simulink model "sf_traffic_light"  (R2025b)
settings: Solver=FixedStepDiscrete  StartTime=0.0  StopTime=1000  FixedStep=0.1  RelTol=1e-3  EnableMultiTasking=on
undefined symbols (not defined in the file or in its folder): greenLightLocked, greenLightRequested
libraries: sf_traffic_light_lib x7
settings Model: Creator=The MathWorks, Inc.  LastModifiedBy=The MathWorks, Inc.
settings SolverCC: AlgebraicLoopSolver=TrustRegion
settings DataIOCC: LimitDataPoints=on  SaveFormat=Array  ReturnWorkspaceOutputs=off
settings OptimizationCC: ReuseModelBlockBuffer=off  ExpressionDepthLimit=2147483647.0  InitFltsAndDblsToZero=on  EfficientMapNaN2IntZero=off  LifeSpan=inf
settings DebuggingCC: SaveWithParameterizedLinksMsg=none  UnderspecifiedInitializationDetection=Classic  MergeDetectMultiDrivingBlocksExec=none  SignalResolutionControl=TryResolveAllWithWarning  SolverPrmCheckMsg=warning  MultiTaskDSMMsg=warning  MultiTaskCondExecSysMsg=none  FcnCallInpInsideContextMsg=warning  UnconnectedInputMsg=warning  UnconnectedOutputMsg=warning  UnconnectedLineMsg=warning  StateNameClashWarn=warning  SFUnexpectedBacktrackingDiag=warning  SFNoUnconditionalDefaultTransitionDiag=warning  SFExecutionAtInitializationDiag=none  ArithmeticOperatorsInVariantConditions=warning
settings HardwareCC: ProdBitPerPointer=32.0  ProdBitPerSizeT=32.0  ProdBitPerPtrDiffT=32.0  ProdLargestAtomicFloat=None  ProdIntDivRoundTo=Undefined  ProdEndianess=Unspecified  ProdWordSize=32.0  ProdHWDeviceType=32-bit Generic
settings ModelReferenceCC: EnableRefExpFcnMdlSchedulingChecks=on  PropagateSignalLabelsOutOfModel=off
settings SFSimCC: SimUseLocalCustomCode=off  SimParseCustomCode=off  CustomCodeUndefinedFunction=UseInterfaceOnly
settings RTWCC: RTWUseLocalCustomCode=off  GPUComputeCapability=3.5
settings CodeAppCC: StateflowObjectComments=on
settings GRTTargetCC: TargetFcnLib=ansi_tfl_tmw.mat  TargetLangStandard=C89/C90 (ANSI)  CombineOutputUpdateFcns=off  GRTInterface=on
settings ConfigComp: CovMetricSettings=dw  CovSaveCumulativeToWorkspaceVar=on  CovSaveSingleToWorkspaceVar=on  CovExternalEMLEnable=off  CovSFcnEnable=off

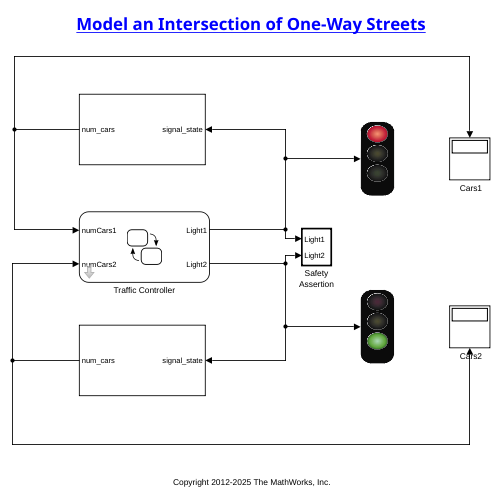
[thumbnail: Simulink's stored preview of the top-level diagram]
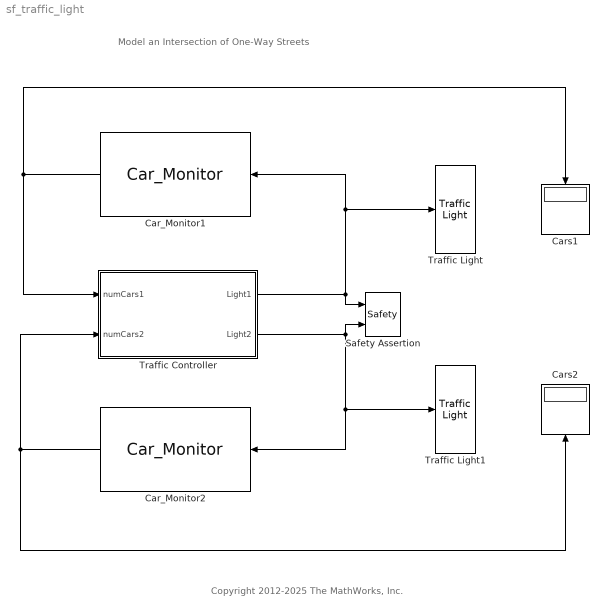
== system sf_traffic_light ==
  note: Copyright 2012-2025 The MathWorks, Inc.
  note: Model an Intersection of One-Way Streets
  " Cars1" : Display
  " Cars2" : Display
  Car_Monitor1 : sf_traffic_light_lib/Car_Monitor  SystemSampleTime=-1  VariantActivationTime=update diagram  EmptyChoice=off  PassThrough=off  PassThroughVariantControl=(default)  EmptyChoiceVariantControl=(default)  AllowFlexibleInterface=on  Latency=0  AutoFrameSizeCalculation=off
  Car_Monitor2 : sf_traffic_light_lib/Car_Monitor  SystemSampleTime=-1  VariantActivationTime=update diagram  EmptyChoice=off  PassThrough=off  PassThroughVariantControl=(default)  EmptyChoiceVariantControl=(default)  AllowFlexibleInterface=on  Latency=0  AutoFrameSizeCalculation=off
  Safety Assertion : sf_traffic_light_lib/Safety  SystemSampleTime=-1  VariantActivationTime=update diagram  EmptyChoice=off  PassThrough=off  PassThroughVariantControl=(default)  EmptyChoiceVariantControl=(default)  AllowFlexibleInterface=on  Latency=0  AutoFrameSizeCalculation=off
  Traffic Controller : Stateflow chart  TreatAsAtomicUnit=on  mask{REDDELAY=6, YELLOWDELAY=15, GREENDELAY=180, MINGREENDELAY=120, MAXREDDELAY=360}
  Traffic Light : sf_traffic_light_lib/Traffic Light  mode=LightModeType.Red
  Traffic Light1 : sf_traffic_light_lib/Traffic Light  mode=LightModeType.Green
  wires:
  Car_Monitor2/1 -> Traffic Controller/2(numCars2), " Cars2"/1
  Car_Monitor1/1 -> Traffic Controller/1(numCars1), " Cars1"/1
  Traffic Controller/2(Light2) -> Safety Assertion/2, Traffic Light1/1, Car_Monitor2/1
  Traffic Controller/1(Light1) -> Car_Monitor1/1, Traffic Light/1, Safety Assertion/1

== stateflow chart sf_traffic_light/Traffic Controller ==
  state Controller
    state Light1Controller [parallel]
      settings: executionOrder=1
    state Light2Controller [parallel]
      settings: executionOrder=2
  data: numCars1 input; numCars2 input; GREENDELAY parameter; MAXREDDELAY parameter; REDDELAY parameter; YELLOWDELAY parameter; MINGREENDELAY parameter; Light1 output Enum: LightModeType; greenLightLocked local boolean; greenLightRequested local boolean; Light2 output Enum: LightModeType
